simulink model "RW_3Axis_Control"  (R2026b)
settings: Solver=ode45  StopTime=10  MaxStep=0.001  RelTol=1e-8
model workspace (MAT data in the model file):
  Ja = [0.001  0  0; 0  0.001  0; 0  0  0.001]
  Jsc = [0.2  0.01  -0.005; 0.01  0.25  0.008; -0.005  0.008  0.3]
  wn = 1
  zeta = 1
libraries: aerolibutil x1
settings Model: Creator=송성혁  LastModifiedBy=송성혁

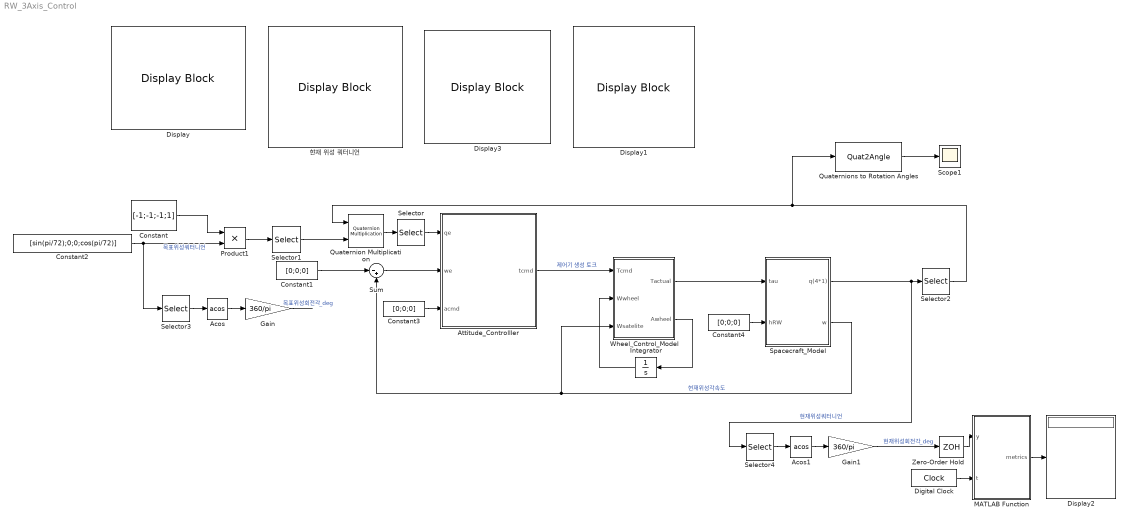
== system RW_3Axis_Control ==
  Acos : Trigonometry  Operator=acos
  Acos1 : Trigonometry  Operator=acos
  Attitude_Controlller : Subsystem
  Constant : Constant  Value=[-1;-1;-1;1]
  Constant1 : Constant  Value=[0;0;0]
  Constant2 : Constant  Value=[sin(pi/72);0;0;cos(pi/72)]
  Constant3 : Constant  Value=[0;0;0]
  Constant4 : Constant  Value=[0;0;0]
  Digital Clock : DigitalClock  SampleTime=0.001
  Display : DisplayBlock  LabelPosition=Bottom  Transparency=1  GridColor=[0.502, 0.502, 0.502]
  Display1 : DisplayBlock  LabelPosition=Bottom  Format=long  Transparency=1  GridColor=[0.502, 0.502, 0.502]
  Display2 : Display
  Display3 : DisplayBlock  LabelPosition=Bottom  Transparency=1  GridColor=[0.502, 0.502, 0.502]
  Gain : Gain  Gain=360/pi
  Gain1 : Gain  Gain=360/pi
  Integrator : Integrator  InitialCondition=[0;0;0]
  MATLAB Function : MATLAB Function  TreatAsAtomicUnit=on
  Product1 : Product
  Quaternion Multiplication : aerolibutil/Quaternion Multiplication
  Quaternions to Rotation Angles : Quat2Angle
      settings: AttributesFormatString=Rotation Order: %<rotationOrder>
  Scope1 : Scope
      settings: ActiveDisplayYMinimum=-0.01090285694316852  ActiveDisplayYMaximum=0.098125712488516689  DataLoggingVariableName=ScopeData3
  Selector : Selector  InputPortWidth=4  IndexOptions=Index vector (dialog)  Indices=[2 3 4]  OutputSizes=1
  Selector1 : Selector  InputPortWidth=4  IndexOptions=Index vector (dialog)  Indices=[4 1 2 3]  OutputSizes=1
  Selector2 : Selector  InputPortWidth=4  IndexOptions=Index vector (dialog)  Indices=[4 1 2 3]  OutputSizes=1
  Selector3 : Selector  InputPortWidth=4  IndexOptions=Index vector (dialog)  Indices=[4]  OutputSizes=1
  Selector4 : Selector  InputPortWidth=4  IndexOptions=Index vector (dialog)  Indices=[4]  OutputSizes=1
  Spacecraft_Model : Subsystem
  Sum : Sum  Inputs=|-+
  Wheel_Control_Model : Subsystem
  Zero-Order Hold : ZeroOrderHold  SampleTime=0.001
  햔재 위성 쿼터니언 : DisplayBlock  LabelPosition=Bottom  Format=long  Transparency=1  GridColor=[0.502, 0.502, 0.502]
  wires:
  Spacecraft_Model/2(w) -> Wheel_Control_Model/3(Wsatelite), Sum/2  "현재위성각속도"
  Constant/1 -> Product1/1
  Constant2/1 -> Selector3/1, Product1/2  "목표위성쿼터니언"
  Constant1/1 -> Sum/1
  Attitude_Controlller/1(tcmd) -> Wheel_Control_Model/1(Tcmd)  "제어기 생성 토크"
  Constant4/1 -> Spacecraft_Model/2(hRW)
  Quaternions to Rotation Angles/1 -> Scope1/1
  Quaternion Multiplication/1 -> Selector/1
  Spacecraft_Model/1(q(4*1)) -> Selector4/1, Selector2/1  "현재위성쿼터니언"
  Selector2/1 -> Quaternion Multiplication/1, Quaternions to Rotation Angles/1
  Product1/1 -> Selector1/1
  Selector1/1 -> Quaternion Multiplication/2
  Selector/1 -> Attitude_Controlller/1(qe)
  Constant3/1 -> Attitude_Controlller/3(acmd)
  Sum/1 -> Attitude_Controlller/2(we)
  Selector3/1 -> Acos/1
  Acos/1 -> Gain/1
  Gain/1 -> ?  "목표위성회전각_deg"
  Acos1/1 -> Gain1/1
  Selector4/1 -> Acos1/1
  Gain1/1 -> Zero-Order Hold/1  "현재위성회전각_deg"
  Zero-Order Hold/1 -> MATLAB Function/1(y)
  Digital Clock/1 -> MATLAB Function/2(t)
  MATLAB Function/1(metrics) -> Display2/1
  Wheel_Control_Model/1(Tactual) -> Spacecraft_Model/1(tau)
  Wheel_Control_Model/2(Awheel) -> Integrator/1
  Integrator/1 -> Wheel_Control_Model/2(Wwheel)

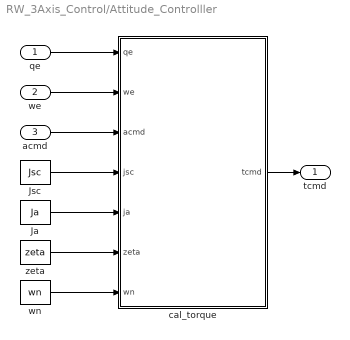
== system RW_3Axis_Control/Attitude_Controlller ==
  qe : Inport
  we : Inport  Port=2
  acmd : Inport  Port=3
  Ja : Constant  Value=Ja
  Jsc : Constant  Value=Jsc
  cal_torque : MATLAB Function  TreatAsAtomicUnit=on
  wn : Constant  Value=wn
  zeta : Constant  Value=zeta
  tcmd : Outport
  wires:
  acmd/1 -> cal_torque/3(acmd)
  qe/1 -> cal_torque/1(qe)
  we/1 -> cal_torque/2(we)
  cal_torque/1(tcmd) -> tcmd/1
  Ja/1 -> cal_torque/5(ja)
  Jsc/1 -> cal_torque/4(jsc)
  zeta/1 -> cal_torque/6(zeta)
  wn/1 -> cal_torque/7(wn)

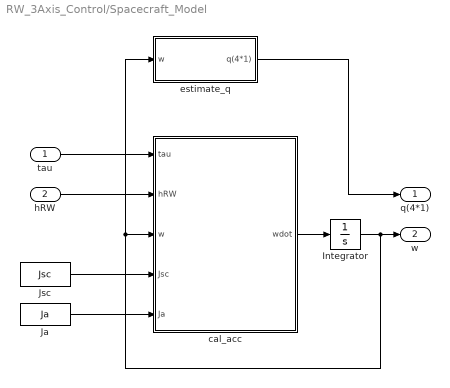
== system RW_3Axis_Control/Spacecraft_Model ==
  tau : Inport
  hRW : Inport  Port=2
  Integrator : Integrator  InitialCondition=[0;0;0]
  Ja : Constant  Value=Ja
  Jsc : Constant  Value=Jsc
  cal_acc : MATLAB Function  TreatAsAtomicUnit=on
  estimate_q : Subsystem
  q(4*1) : Outport
  w : Outport  Port=2
  wires:
  Integrator/1 -> w/1, estimate_q/1(w), cal_acc/3(w)
  cal_acc/1(wdot) -> Integrator/1
  tau/1 -> cal_acc/1(tau)
  hRW/1 -> cal_acc/2(hRW)
  Jsc/1 -> cal_acc/4(Jsc)
  Ja/1 -> cal_acc/5(Ja)
  estimate_q/1(q(4*1)) -> q(4*1)/1

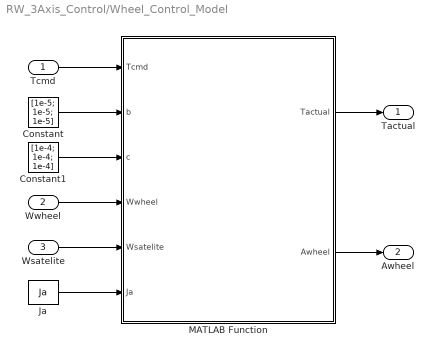
== system RW_3Axis_Control/Wheel_Control_Model ==
  Tcmd : Inport
  Wwheel : Inport  Port=2
  Wsatelite : Inport  Port=3
  Constant : Constant  Value=[1e-5; 1e-5; 1e-5]
  Constant1 : Constant  Value=[1e-4; 1e-4; 1e-4]
  Ja : Constant  Value=Ja
  MATLAB Function : MATLAB Function  TreatAsAtomicUnit=on
  Tactual : Outport
  Awheel : Outport  Port=2
  wires:
  Tcmd/1 -> MATLAB Function/1(Tcmd)
  Wsatelite/1 -> MATLAB Function/5(Wsatelite)
  Wwheel/1 -> MATLAB Function/4(Wwheel)
  MATLAB Function/2(Awheel) -> Awheel/1
  MATLAB Function/1(Tactual) -> Tactual/1
  Constant1/1 -> MATLAB Function/3(c)
  Constant/1 -> MATLAB Function/2(b)
  Ja/1 -> MATLAB Function/6(Ja)

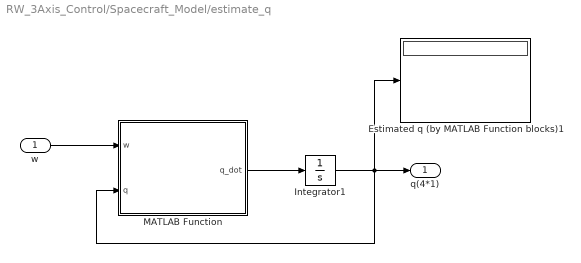
== system RW_3Axis_Control/Spacecraft_Model/estimate_q ==
  w : Inport
  Estimated q (by MATLAB Function blocks)1 : Display
  Integrator1 : Integrator  InitialCondition=[0; 0; 0; 1]
  MATLAB Function : MATLAB Function  TreatAsAtomicUnit=on
  q(4*1) : Outport
  wires:
  w/1 -> MATLAB Function/1(w)
  MATLAB Function/1(q_dot) -> Integrator1/1
  Integrator1/1 -> q(4*1)/1, Estimated q (by MATLAB Function blocks)1/1, MATLAB Function/2(q)

== matlab function RW_3Axis_Control/MATLAB Function ==
  data: y input; metrics output; t input

function metrics = fcn(y, t)

target = 5;           % 목표 자세 [deg]
low = 0.1 * target;
high = 0.9 * target;
band = 0.02 * target;

persistent t10 t90 settle_t ymax was_inside

if isempty(t10)
    t10 = -1;
    t90 = -1;
    settle_t = -1;
    ymax = 0;
    was_inside = false;
end

% 1. 상승시간
if t10 < 0 && y >= low
    t10 = t;
end

if t90 < 0 && y >= high
    t90 = t;
end

Tr = -1;

if t10 >= 0 && t90 >= 0
    Tr = t90 - t10;
end

% 2. 정착시간 (2%)
inside = abs(target - y) <= band;

if inside && ~was_inside
    settle_t = t;
end

if ~inside
    settle_t = -1;
end

was_inside = inside;
Ts = settle_t;

% 3. 오버슈트
ymax = max(ymax, y);
OS = max(0, (ymax - target) / target * 100);

% 4. 현재 자세 오차
error_deg = target - y;

% 5. 감쇠비 및 고유진동수 추정
zeta = -1;
wn = -1;

if OS > 0 && OS < 100 && Ts > 0
    Mp = OS / 100;
    L = log(Mp);

    zeta = -L / sqrt(pi^2 + L^2);
    wn = 4 / (zeta * Ts);
end

% 6. 하나의 열벡터로 출력
metrics = [Tr;
    Ts;
    OS;
    error_deg;
    zeta;
    wn];

end

== matlab function RW_3Axis_Control/Spacecraft_Model/cal_acc ==
  data: tau input; wdot output; hRW input; w input; Jsc input; Ja input

function wdot = cal_acc(tau, hRW, w, Jsc, Ja)
%#codegen

% 유효 관성행렬
Jeff = Jsc - Ja;

% 전체 각운동량
H = Jsc*w + hRW;

% 위성 각가속도
wdot = Jeff \ (cross(H,w) + tau);%tau = -Tm = 위성에 가하는 토크

end

== matlab function RW_3Axis_Control/Wheel_Control_Model/MATLAB Function ==
  data: Tcmd input; Tactual output; b input; c input; Wwheel input; Wsatelite input; Awheel output; Ja input
function [Tactual, Awheel]= fcn(Tcmd, b, c, Wwheel, Wsatelite, Ja)

w_w = Wwheel - Wsatelite;%w_w=휠_상대각속도  Wwheel=휠_절대각속도
w_eps = 0.1; % rad/s, 시험용 평활화 계수
Tf = b .* w_w + c .* tanh(w_w ./ w_eps);

Tactual = Tcmd + Tf;%Tactual=실제위성에 적용되는 토크

Tw = -Tactual;%Tw=모터_순토크 
Awheel = Ja\(Tw);

end

== matlab function RW_3Axis_Control/Attitude_Controlller/cal_torque ==
  data: qe input; tcmd output; we input; acmd input; jsc input; ja input; zeta input; wn input
function tcmd = cal_torque(qe, we, acmd, jsc, ja, zeta, wn)

kp = 2*wn^2*(jsc-ja);
kd = 2*zeta*wn*(jsc-ja);

tcmd = -kp*qe - kd*we + (jsc-ja)*acmd;

end

== matlab function RW_3Axis_Control/Spacecraft_Model/estimate_q/MATLAB Function ==
  data: w input; q input; q_dot output

function q_dot = fcn(w, q)

wx = w(1);
wy = w(2);
wz = w(3);

Omega = [  0,   wz, -wy, wx;
    -wz,    0,  wx, wy;
    wy,  -wx,   0, wz;
    -wx,  -wy, -wz,  0];

q_dot = 0.5 * Omega * q;

end
